simulink model "Quad_UAV_Dynamics_R2024a"  (R2024a)
settings: Solver=VariableStepAuto  StartTime=0.0  StopTime=inf  RelTol=1e-3
PreLoadFcn:
  | InitVars;
values from neighbouring files (symbols this model uses):
  dragCoeffMov = diag([0.1, 0.1, 0.2])    [InitVars.m]
  g = 9.80665    [InitVars.m]
  m_to_mm = 1000    [InitVars.m]
  mass = 1.0    (= 1)    [InitVars.m]
  ms2_to_mg = 1000 / g    (= 101.971621298)    [InitVars.m]
  ms_to_cms = 100    [InitVars.m]
  ref_height = 488.0    (= 488)    [InitVars.m]
  ref_lat = 47.397742    [InitVars.m]
  ref_lon = 8.545594    [InitVars.m]
  rotorDir = [-1; -1; 1; 1]    [InitVars.m]
  rotorPositions = [ armLength*cos(pi/4), -armLength*sin(pi/4), 0 ... (first row only)    [InitVars.m]
  rotorThrustMax = 5.0    (= 5)    [InitVars.m]
  rotorTimeConst = 0.05    [InitVars.m]
  rotorTorqueMax = 0.05    [InitVars.m]
  SampleTime = 0.005    [InitVars.m]    (also in px4HostTarget_TCPIP_Read.m = -1)
  windVel = [0; 0; 0]    [InitVars.m]
undefined symbols (not defined in the file or in its folder): contact, control, fractalcoef, Payload, uav
libraries: uavmavlinklib x5, simulink x2, sharedtransform x2, aerolibatmos2 x1, sensorgpslib x1, robotcorelib x1, mspsensorlib x1, shared6dof x1, uavutilslib x1
(part 2 of 2)

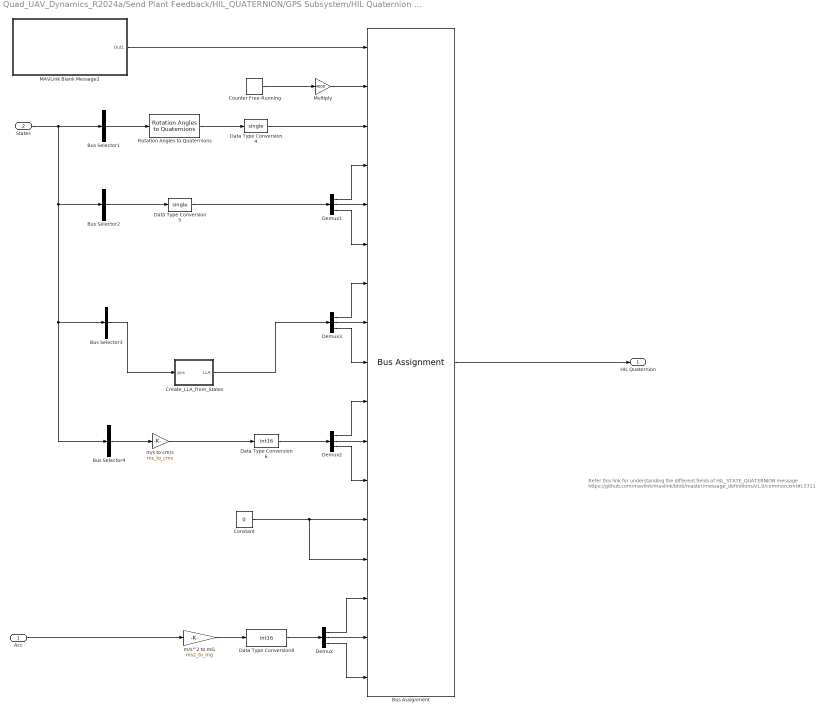
== system Quad_UAV_Dynamics_R2024a/Send Plant Feedback/HIL_QUATERNION/GPS Subsystem/HIL Quaternion Creation Subsystem ==
  note: Refer this link for understanding the different fields of HIL_STATE_QUATERNION message https://github.com/mavlink/mavlink/blob/master/message_definitions/v1.0/common.xml#L5711
  Acc : Inport
  States : Inport  Port=2
  Bus Assignment : BusAssignment  AssignedSignals=Payload.time_usec,Payload.attitude_quaternion,Payload.rollspeed,Payload.pitchspeed,Payload.yawspeed,Payload.lat,Payload.lon,Payload.alt,Payload.vx,Payload.vy,Payload.vz,Payload.ind_airspeed,Payload.true_airspeed,Payload.xacc,Payload.yacc,Payload.zacc
  Bus Selector1 : BusSelector  OutputSignals=yaw,pitch,roll  OutputAsBus=on
  Bus Selector2 : BusSelector  OutputSignals=r,q,p  OutputAsBus=on
  Bus Selector3 : BusSelector  OutputSignals=X,Y,Z  OutputAsBus=on
  Bus Selector4 : BusSelector  OutputSignals=dx,dy,dz  OutputAsBus=on
  Constant : Constant  Value=0  OutDataTypeStr=Inherit: Inherit via back propagation
  Counter Free-Running : simulink/Sources/Counter Free-Running  NumBits=64  tsamp=-1
  Create_LLA_from_States : MATLAB Function  TreatAsAtomicUnit=on
  Data Type Conversion4 : DataTypeConversion  OutDataTypeStr=single  SaturateOnIntegerOverflow=off  RndMeth=Floor
  Data Type Conversion5 : DataTypeConversion  OutDataTypeStr=single  SaturateOnIntegerOverflow=off  RndMeth=Floor
  Data Type Conversion6 : DataTypeConversion  OutDataTypeStr=int16  SaturateOnIntegerOverflow=off  RndMeth=Floor
  Data Type Conversion8 : DataTypeConversion  OutDataTypeStr=int16  SaturateOnIntegerOverflow=off  RndMeth=Floor
  Demux{,1..3} (4 alike) : Demux  Outputs=3
  MAVLink Blank Message2 : Subsystem  InitFcn=uav.sluav.internal.mavlink.util.errorIfBlocksConflict(bdroot(gcb))  mask(MAVLink Blank Message){dialectSource=Select from standard MAVLink dialects, dialect=common.xml, dialectCustom=common.xml, version=2, messageType=HIL_STATE_QUATERNION, SystemID=2, ComponentID=51, SampleTime=SampleTime}
      mask prompts: dialectSource "uav:robotsluav:mavlink:DialectSourcePrompt"; dialect "uav:robotsluav:mavlink:DialectPrompt"; dialectCustom "uav:robotsluav:mavlink:DialectPromptCustom"; version "uav:robotsluav:mavlink:VersionPrompt"; messageType "uav:robotsluav:mavlink:MessageTypePrompt"; SystemID "uav:robotsluav:mavlink:EnterSystemIDPrompt"; ComponentID "uav:robotsluav:mavlink:EnterComponentIDPrompt"; SampleTime "Simulink:blkprm_prompts:AllSrcBlksSampleTime"
      mask help: uav:robotsluav:mavlink:BlankMessageDescription
      mask init:
      | uav.sluav.internal.mavlink.block.MessageBlockMask.dispatch('maskInitialize', gcb)
      settings: LibrarySourceBlock=uavmavlinklib/MAVLink Blank Message  ModelCloseFcn=uav.sluav.internal.mavlink.block.MessageBlockMask.dispatch('modelCloseFcn', gcb);
      mask Help: eval("helpview('uav','uavMAVLinkBlankMessage')");
      mask TypeOptions dialectSource: uav:robotsluav:mavlink:DialectSourceFromStandard | uav:robotsluav:mavlink:DialectSourceSpecifyOwn
      mask Callback dialectSource: uav.sluav.internal.mavlink.block.MessageBlockMask.dispatch('dialectSourceSelect', gcb);
      mask TypeOptions dialect: uav:robotsluav:mavlink:DialectCommon | uav:robotsluav:mavlink:DialectArdupilotmega | uav:robotsluav:mavlink:DialectASLUAV | uav:robotsluav:mavlink:DialectAutoquad | uav:robotsluav:mavlink:DialectIcarous | uav:robotsluav:mavlink:DialectMatrixpilot | uav:robotsluav:mavlink:DialectMinimal | uav:robotsluav:mavlink:DialectPaparazzi | uav:robotsluav:mavlink:DialectSlugs | uav:robotsluav:mavlink:DialectStandard | uav:robotsluav:mavlink:DialectUalberta | uav:robotsluav:mavlink:DialectUAvionix
      mask Callback dialect: uav.sluav.internal.mavlink.block.MessageBlockMask.dispatch('dialectEdit', gcb);
      mask Callback dialectCustom: uav.sluav.internal.mavlink.block.MessageBlockMask.dispatch('dialectEdit', gcb);
      mask TypeOptions version: 2 | 1
      mask Callback version: uav.sluav.internal.mavlink.block.MessageBlockMask.dispatch('versionEdit', gcb);
      mask Callback messageType: uav.sluav.internal.mavlink.block.MessageBlockMask.dispatch('messageTypeEdit', gcb);
      mask Callback SystemID: uav.sluav.internal.mavlink.block.MessageBlockMask.dispatch('updateSystemAndComponentID', gcb);
      mask Callback ComponentID: uav.sluav.internal.mavlink.block.MessageBlockMask.dispatch('updateSystemAndComponentID', gcb);
      mask TypeOptions SampleTime: MsgIDConstant/SampleTime
      mask DialogControl MainContainer Prompt: uav:robotsluav:mavlink:MainTabTitle
      mask DialogControl dialectSource Prompt: MAVLink dialect source:
      mask DialogControl dialect Prompt: MAVLink dialect:
      mask DialogControl dialectCustom Prompt: MAVLink dialect:
      mask DialogControl dialectBrowseButton Prompt: uav:robotsluav:mavlink:DialectBrowsePrompt
      mask DialogControl dialectBrowseButton Callback: uav.sluav.internal.mavlink.block.MessageBlockMask.dispatch('dialectBrowse', gcb);
      mask DialogControl version Prompt: MAVLink version:
      mask DialogControl messageType Prompt: MAVLink message type:
      mask DialogControl msgSelectButton Prompt: uav:robotsluav:mavlink:MessageSelectPrompt
      mask DialogControl msgSelectButton Callback: uav.sluav.internal.mavlink.block.MessageBlockMask.dispatch('messageTypeSelect', gcb, 'uav.sluav.internal.mavlink.dlg.MessageTypeSelector');
      mask DialogControl SystemID Prompt: System ID:
      mask DialogControl ComponentID Prompt: Component ID:
      mask DialogControl SampleTime Prompt: Sample time:
      mask Display:
      | color('black');
      | text(0.83, 0.10, 'HIL_STATE_QUATERNION', 'horizontalAlignment', 'right');
      | port_label('output', 1, 'Msg');
  Multiply : Gain  Gain=4000  OutDataTypeStr=Inherit: Inherit via back propagation
  Rotation Angles to Quaternions : sharedtransform/Rotation Angles to Quaternions  rotationOrder=ZYX  aMode=aMode
  m/s to cm/s : Gain  Gain=ms_to_cms
  m/s^2 to mG : Gain  Gain=ms2_to_mg
  HIL Quaternion : Outport
  wires:
  Counter Free-Running/1 -> Multiply/1
  MAVLink Blank Message2/1(Out1) -> Bus Assignment/1
  Multiply/1 -> Bus Assignment/2
  Bus Assignment/1 -> HIL Quaternion/1
  States/1 -> Bus Selector1/1, Bus Selector2/1, Bus Selector4/1, Bus Selector3/1
  Rotation Angles to Quaternions/1 -> Data Type Conversion4/1
  Data Type Conversion4/1 -> Bus Assignment/3
  Demux/3 -> Bus Assignment/17
  Demux/1 -> Bus Assignment/15
  Demux/2 -> Bus Assignment/16
  Constant/1 -> Bus Assignment/14, Bus Assignment/13
  m/s to cm/s/1 -> Data Type Conversion6/1
  Data Type Conversion6/1 -> Demux2/1
  Demux2/3 -> Bus Assignment/12
  Demux2/2 -> Bus Assignment/11
  Demux2/1 -> Bus Assignment/10
  Demux3/1 -> Bus Assignment/7
  Demux3/2 -> Bus Assignment/8
  Demux3/3 -> Bus Assignment/9
  Data Type Conversion8/1 -> Demux/1
  Acc/1 -> m/s^2 to mG/1
  m/s^2 to mG/1 -> Data Type Conversion8/1
  Bus Selector1/1 -> Rotation Angles to Quaternions/1
  Data Type Conversion5/1 -> Demux1/1
  Demux1/3 -> Bus Assignment/6
  Demux1/2 -> Bus Assignment/5
  Demux1/1 -> Bus Assignment/4
  Bus Selector2/1 -> Data Type Conversion5/1
  Bus Selector3/1 -> Create_LLA_from_States/1(pos)
  Bus Selector4/1 -> m/s to cm/s/1
  Create_LLA_from_States/1(LLA) -> Demux3/1

== system Quad_UAV_Dynamics_R2024a/Send Plant Feedback/HIL_SENSOR/Hil Sensor Creation subsystem/MAVLink Blank Message1 ==
  ComponentIDConstant : Constant  Value=51  OutDataTypeStr=uint8  SampleTime=-1
  MAVLinkMsgBusCreator : BusCreator  Inputs=5  OutDataTypeStr=Bus: SL_Bus_MAVLink_HIL_SENSOR_Packet  NonVirtualBus=on
  MsgIDConstant : Constant  Value=107  OutDataTypeStr=uint32  SampleTime=SampleTime
  MsgModifier : MATLABSystem  System=uav.sluav.internal.system.MAVLinkMsgModifier  SLBusName=SL_Bus_MAVLink_HIL_SENSOR_Payload
      mask Type: uav.sluav.internal.system.MAVLinkMsgModifier
      mask Display:
      | disp('MAVLinkMsgModifier');
      | port_label('input',1,'msgID');
      | port_label('input',2,'inputBusStruct');
      | port_label('output',1,'modifiedBusStruct');
  PayloadConstant : Constant  Value=0  OutDataTypeStr=Bus: SL_Bus_MAVLink_HIL_SENSOR_Payload  SampleTime=-1
  SequenceConstant : Constant  Value=0  OutDataTypeStr=uint8  SampleTime=-1
  SystemIDConstant : Constant  Value=2  OutDataTypeStr=uint8  SampleTime=-1
  Out1 : Outport
  wires:
  MsgModifier/1 -> MAVLinkMsgBusCreator/5  "Payload"
  MAVLinkMsgBusCreator/1 -> Out1/1
  MsgIDConstant/1 -> MsgModifier/1, MAVLinkMsgBusCreator/1  "MsgID"
  SystemIDConstant/1 -> MAVLinkMsgBusCreator/2  "SystemID"
  ComponentIDConstant/1 -> MAVLinkMsgBusCreator/3  "ComponentID"
  SequenceConstant/1 -> MAVLinkMsgBusCreator/4  "Sequence"
  PayloadConstant/1 -> MsgModifier/2  "Payload"

== system Quad_UAV_Dynamics_R2024a/Core plant/Quadcopter model/Force and Moment Calculation/Ground Model/Friction Force ==
  V : Inport
  Fn : Inport  Port=2
  Product : Product
  Saturation : Saturate  UpperLimit=contact.translation.maxFriction  LowerLimit=-contact.translation.maxFriction
  Soft Coulomb Friction : Subsystem
  Unary Minus : UnaryMinus
  Friction : Outport
  wires:
  Fn/1 -> Product/2
  Soft Coulomb Friction/1(Out1) -> Product/1
  Product/1 -> Unary Minus/1
  V/1 -> Soft Coulomb Friction/1(In1)
  Unary Minus/1 -> Saturation/1
  Saturation/1 -> Friction/1

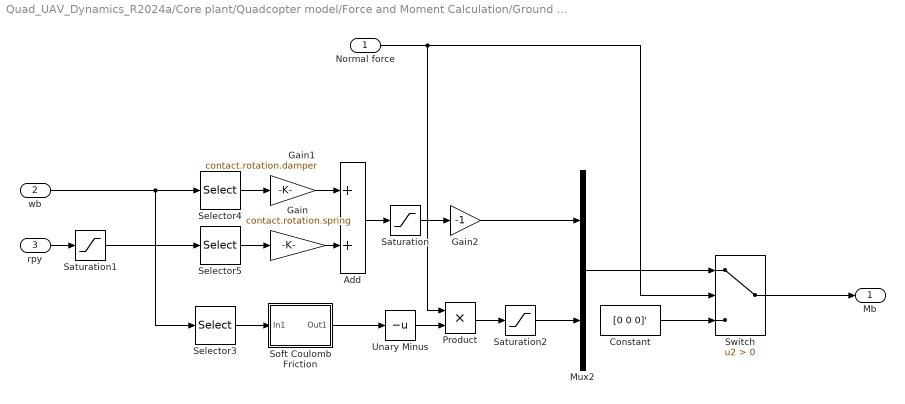
== system Quad_UAV_Dynamics_R2024a/Core plant/Quadcopter model/Force and Moment Calculation/Ground Model/Ground Moment Model ==
  Normal force : Inport
  wb : Inport  Port=2
  rpy : Inport  Port=3
  Add : Sum
  Constant : Constant  Value=[0 0 0]'
  Gain : Gain  Gain=contact.rotation.spring
  Gain1 : Gain  Gain=contact.rotation.damper
  Gain2 : Gain  Gain=-1
  Mux2 : Mux  Inputs=2
  Product : Product
  Saturation : Saturate  UpperLimit=control.rotation.maxMoment  LowerLimit=-control.rotation.maxMoment
  Saturation1 : Saturate  UpperLimit=20*pi/180  LowerLimit=-20*pi/180
  Saturation2 : Saturate  UpperLimit=control.rotation.maxMoment  LowerLimit=-control.rotation.maxMoment
  Selector3 : Selector  InputPortWidth=3  IndexOptions=Index vector (dialog)  Indices=[3]  OutputSizes=1
  Selector4 : Selector  InputPortWidth=3  IndexOptions=Index vector (dialog)  Indices=[1, 2]  OutputSizes=1
  Selector5 : Selector  InputPortWidth=3  IndexOptions=Index vector (dialog)  Indices=[1, 2]  OutputSizes=1
  Soft Coulomb Friction : Subsystem
  Switch : Switch  Criteria=u2 > Threshold  SaturateOnIntegerOverflow=off  InputSameDT=off
  Unary Minus : UnaryMinus
  Mb : Outport
  wires:
  Gain2/1 -> Mux2/1
  Add/1 -> Saturation/1
  Gain/1 -> Add/2
  Saturation/1 -> Gain2/1
  Selector4/1 -> Gain1/1
  Gain1/1 -> Add/1
  Constant/1 -> Switch/3
  Selector5/1 -> Gain/1
  Switch/1 -> Mb/1
  Mux2/1 -> Switch/1
  Normal force/1 -> Product/1, Switch/2
  rpy/1 -> Saturation1/1
  Saturation1/1 -> Selector5/1
  wb/1 -> Selector4/1, Selector3/1
  Selector3/1 -> Soft Coulomb Friction/1(In1)
  Soft Coulomb Friction/1(Out1) -> Unary Minus/1
  Unary Minus/1 -> Product/2
  Product/1 -> Saturation2/1
  Saturation2/1 -> Mux2/2

== system Quad_UAV_Dynamics_R2024a/Core plant/Quadcopter model/Force and Moment Calculation/Ground Model/Normal Force ==
  Vz : Inport
  Z : Inport  Port=2
  Add : Sum
  Constant : Constant  Value=0
  Damper Kp : Gain  Gain=-contact.translation.damper
  Saturation : Saturate  UpperLimit=contact.translation.maxNormal  LowerLimit=0
  Spring Kp : Gain  Gain=-contact.translation.spring
  Switch : Switch  Criteria=u2 > Threshold  SaturateOnIntegerOverflow=off  InputSameDT=off
  Unary Minus : UnaryMinus
  Unary Minus1 : UnaryMinus
  Normal : Outport
  wires:
  Constant/1 -> Switch/1
  Z/1 -> Unary Minus/1
  Switch/1 -> Saturation/1
  Damper Kp/1 -> Add/2
  Add/1 -> Switch/3
  Spring Kp/1 -> Add/1
  Vz/1 -> Unary Minus1/1
  Saturation/1 -> Normal/1
  Unary Minus/1 -> Spring Kp/1, Switch/2
  Unary Minus1/1 -> Damper Kp/1

== system Quad_UAV_Dynamics_R2024a/Core plant/Quadcopter model/Force and Moment Calculation/Rotor Model/Thrust model ==
  In1 : Inport
  Demux : Demux
  Mux : Mux
  Transfer Fcn{,2..4} (4 alike) : TransferFcn  Numerator=[rotorThrustMax]  Denominator=[rotorTimeConst 1]
  Out1 : Outport
  wires:
  Transfer Fcn3/1 -> Mux/2
  Demux/1 -> Transfer Fcn4/1
  Transfer Fcn2/1 -> Mux/3
  Demux/3 -> Transfer Fcn2/1
  Mux/1 -> Out1/1
  Transfer Fcn4/1 -> Mux/1
  Demux/4 -> Transfer Fcn/1
  Demux/2 -> Transfer Fcn3/1
  Transfer Fcn/1 -> Mux/4
  In1/1 -> Demux/1

== system Quad_UAV_Dynamics_R2024a/Core plant/Quadcopter model/Force and Moment Calculation/Rotor Model/Torque model ==
  In1 : Inport
  Demux : Demux
  Mux : Mux
  Transfer Fcn{1..4} (4 alike) : TransferFcn  Numerator=[rotorTorqueMax]  Denominator=[rotorTimeConst 1]
  Out1 : Outport
  wires:
  Transfer Fcn4/1 -> Mux/4
  Demux/1 -> Transfer Fcn1/1
  Transfer Fcn3/1 -> Mux/3
  Transfer Fcn2/1 -> Mux/2
  Demux/2 -> Transfer Fcn2/1
  Demux/4 -> Transfer Fcn4/1
  Demux/3 -> Transfer Fcn3/1
  Mux/1 -> Out1/1
  Transfer Fcn1/1 -> Mux/1
  In1/1 -> Demux/1

== system Quad_UAV_Dynamics_R2024a/Send Plant Feedback/HIL_QUATERNION/GPS Subsystem/HIL Quaternion Creation Subsystem/MAVLink Blank Message2 ==
  ComponentIDConstant : Constant  Value=51  OutDataTypeStr=uint8  SampleTime=-1
  MAVLinkMsgBusCreator : BusCreator  Inputs=5  OutDataTypeStr=Bus: SL_Bus_MAVLink_HIL_STATE_QUATERNION_Packet  NonVirtualBus=on
  MsgIDConstant : Constant  Value=115  OutDataTypeStr=uint32  SampleTime=SampleTime
  MsgModifier : MATLABSystem  System=uav.sluav.internal.system.MAVLinkMsgModifier  SLBusName=SL_Bus_MAVLink_HIL_STATE_QUATERNION_Payload
      mask Type: uav.sluav.internal.system.MAVLinkMsgModifier
      mask Display:
      | disp('MAVLinkMsgModifier');
      | port_label('input',1,'msgID');
      | port_label('input',2,'inputBusStruct');
      | port_label('output',1,'modifiedBusStruct');
  PayloadConstant : Constant  Value=0  OutDataTypeStr=Bus: SL_Bus_MAVLink_HIL_STATE_QUATERNION_Payload  SampleTime=-1
  SequenceConstant : Constant  Value=0  OutDataTypeStr=uint8  SampleTime=-1
  SystemIDConstant : Constant  Value=2  OutDataTypeStr=uint8  SampleTime=-1
  Out1 : Outport
  wires:
  MsgModifier/1 -> MAVLinkMsgBusCreator/5  "Payload"
  MAVLinkMsgBusCreator/1 -> Out1/1
  MsgIDConstant/1 -> MsgModifier/1, MAVLinkMsgBusCreator/1  "MsgID"
  SystemIDConstant/1 -> MAVLinkMsgBusCreator/2  "SystemID"
  ComponentIDConstant/1 -> MAVLinkMsgBusCreator/3  "ComponentID"
  SequenceConstant/1 -> MAVLinkMsgBusCreator/4  "Sequence"
  PayloadConstant/1 -> MsgModifier/2  "Payload"

== system Quad_UAV_Dynamics_R2024a/Core plant/Quadcopter model/Force and Moment Calculation/Ground Model/Friction Force/Soft Coulomb Friction ==
  note: Pennestrì, E., Rossi, V., Salvini, P. et al. Review and comparison of dry friction force models. Nonlinear Dyn 83, 1785–1801 (2016). https://doi.org/10.1007/s11071-015-2485-3
  In1 : Inport
  Tanh : Trigonometry  Operator=tanh
  friction coefficient : Gain  Gain=contact.translation.friction
  vd : Gain  Gain=1/contact.translation.vd
  Out1 : Outport
  wires:
  In1/1 -> vd/1
  vd/1 -> Tanh/1
  Tanh/1 -> friction coefficient/1
  friction coefficient/1 -> Out1/1

== system Quad_UAV_Dynamics_R2024a/Core plant/Quadcopter model/Force and Moment Calculation/Ground Model/Ground Moment Model/Soft Coulomb Friction ==
  note: Pennestrì, E., Rossi, V., Salvini, P. et al. Review and comparison of dry friction force models. Nonlinear Dyn 83, 1785–1801 (2016). https://doi.org/10.1007/s11071-015-2485-3
  In1 : Inport
  Tanh : Trigonometry  Operator=tanh
  friction coefficient : Gain  Gain=control.rotation.friction
  vd : Gain  Gain=1/control.rotation.vd
  Out1 : Outport
  wires:
  In1/1 -> vd/1
  vd/1 -> Tanh/1
  Tanh/1 -> friction coefficient/1
  friction coefficient/1 -> Out1/1

== matlab function Quad_UAV_Dynamics_R2024a/Send Plant Feedback/HIL_QUATERNION/GPS Subsystem/HIL Quaternion Creation Subsystem/Create_LLA_from_States ==
  data: pos input; LLA output
function LLA = fcn(pos)
% Extract X (North), Y (East), Z (Down) in meters
if isstruct(pos)
    x = pos.X;
    y = pos.Y;
    z = pos.Z;
else
    x = pos(1);
    y = pos(2);
    z = pos(3);
end

% Reference coordinates (from InitVars)
ref_lat = 47.397742;  % Latitude (deg)
ref_lon = 8.545594;   % Longitude (deg)
ref_alt = 488.0;      % Altitude (m)
R_earth = 6378137.0;  % WGS84 Earth radius (m)

% Convert local NED to geodetic LLA
lat = ref_lat + (x / R_earth) * (180 / pi);
lon = ref_lon + (y / (R_earth * cos(ref_lat * pi / 180))) * (180 / pi);
alt = ref_alt - z;

% MAVLink HIL_STATE_QUATERNION scaling: degE7 and mm
lat_e7 = int32(lat * 1e7);
lon_e7 = int32(lon * 1e7);
alt_mm = int32(alt * 1000);

LLA = [lat_e7; lon_e7; alt_mm];

== matlab function Quad_UAV_Dynamics_R2024a/Core plant/Quadcopter model/Force and Moment Calculation/Aerodynamic drag/calcDragVector ==
  data: airVel input; dragVec output; dragCoeff input
function dragVec = fcn(airVel, dragCoeff)

dragVec = dragCoeff * norm(airVel) * airVel;

end

== matlab function Quad_UAV_Dynamics_R2024a/Core plant/Quadcopter model/Force and Moment Calculation/Rotor Model/MATLAB Function ==
  data: thrustEachRotor input; tauEachRotor input; rotorPositions input; netF output; netM output; rotorDir input
function [netF, netM] = getForceMoment(thrustEachRotor, tauEachRotor, rotorPositions, rotorDir)
%#codegen
Fx = 0;
Fy = 0;
Fz = -sum(thrustEachRotor);

netF = [Fx; Fy; Fz];

netM = [0; 0; 0]; %initialize
    for i = 1:4
        rotPos = rotorPositions(:, i);
        Fi = [0, 0, -thrustEachRotor(i)]';
        netM = netM +  cross(rotPos, Fi);%contribution from thrusts of each propeller
        netM(3) = netM(3) - rotorDir(i)*tauEachRotor(i); %contribution from counter torque acting on propeller
    end

end
